simulink model "rocket_launch"  (R2024a)
settings: Solver=FixedStepAuto  StartTime=0.0001  StopTime=140  FixedStep=0.0001  RelTol=1e-3
undefined symbols (not defined in the file or in its folder): deg, Earth, rad, s, WGS84
libraries: aerolibconvert2 x26, matrix_library x5, eePwmGenerator x4, slpidlib x4, aerolibasang x2, sharedtransform x1, simulink x1, aerolibtransform2 x1, shared6dof x1
(part 2 of 2)

== matlab function rocket_launch/AeroDynamics/MATLAB Function3 ==
  data: alpha input; CD output; mach input; delta_e input; CL output; CY output; Cl output; Cm output; delta_a input; delta_r input; b input; p input; q input; r input; V input; Cn output
function [CD,CL,CY,Cl,Cm,Cn]= aeroCoeffs(alpha, mach, delta_e, delta_a, delta_r , b, p, q, r, V)

% 气动系数
CL_0 = -0.404;
CL_alpha = 0.0699;
CL_delE = 0.0026;

CD_0 = -0.239;
CD_alpha = 0.035;
CD_delE = 0.0021;

CY_delR = 0.0039;

Cl_delA = 0.0023;
Cl_delR = 0.0028;
Cl_r = 0.2201;

Cm_0 = -0.0151;
Cm_alpha = 0.0117;
Cm_delE = -0.008;
Cm_q = 0.417;

Cn_delA = 4.997e-4;
Cn_delR = 0.0041;
Cn_p = 0.142;
% 
% % 气动力系数
CL = CL_0 + CL_alpha * alpha + CL_delE * delta_e;
CD = CD_0 + CD_delE * delta_e + CD_alpha * alpha;   % 待补充
CY = CY_delR * delta_r;
% 
% % 气动力矩系数
% Cl = Cl_delA * delta_a + Cl_delR * delta_r + Cl_r * (r*b/(2*V));
% Cm = Cm_0 + Cm_alpha * alpha + Cm_delE * delta_e + Cm_q * (q*b/(2*V));
% Cn = Cn_delA * delta_a + Cn_delR * delta_r + Cn_p * (p*b/(2*V));



end
